simulink model "chbtask"  (R2024b)
settings: Solver=FixedStepDiscrete  StartTime=0.0  StopTime=0.2  FixedStep=5e-5  RelTol=1e-3
values from neighbouring files (symbols this model uses):
  CHB_MODE : value not decoded    [CHB_Data.sldd]
  INV120_CUURENTLOOP_KP = 2.0    [CHB_Data.sldd]
  INV120_CUURENTLOOP_KR = 5.0    [CHB_Data.sldd]
  INV120_VOLTAGELOOP_KI = 0.005    [CHB_Data.sldd]
  INV120_VOLTAGELOOP_KP = 0.5    [CHB_Data.sldd]
  INV240_VOLTAGELOOP_KI = 0.005    [CHB_Data.sldd]
  INV240_VOLTAGELOOP_KP = 0.5    [CHB_Data.sldd]
  PFC120_CUURENTLOOP_KP = 30.0    [CHB_Data.sldd]
  PFC120_CUURENTLOOP_KR = 8.0    [CHB_Data.sldd]
  PFC120_POWERLOOP_KI = 0.0001    [CHB_Data.sldd]
  PFC120_POWERLOOP_KP = 0.005    [CHB_Data.sldd]
  PFC240_CUURENTLOOP_KP = 5.0    [CHB_Data.sldd]
  PFC240_CUURENTLOOP_KR = 10.0    [CHB_Data.sldd]
  PFC240_POWERLOOP_KI = 0.0001    [CHB_Data.sldd]
  PFC240_POWERLOOP_KP = 0.005    [CHB_Data.sldd]
undefined symbols (not defined in the file or in its folder): Ii_rms, Io_rms, Io_rms_a, Io_rms_b, Vi_freq, Vi_rms, Vo_freq, Vo_freq_a, Vo_freq_b, Vo_rms, Vo_rms_a, Vo_rms_b
(part 1 of 3)
settings Model: DataDictionary=CHB_Data.sldd  Creator=licuiting  LastModifiedBy=licuiting
settings OptimizationCC: DefaultParameterBehavior=Inlined  ZeroExternalMemoryAtStartup=off  ZeroInternalMemoryAtStartup=off  OptimizeBlockOrder=speed  DifferentSizesBufferReuse=on  EfficientTunableParamExpr=on
settings DebuggingCC: ParameterTunabilityLossMsg=error
settings HardwareCC: ProdBitPerPointer=32  ProdBitPerSizeT=32  ProdBitPerPtrDiffT=32  ProdLargestAtomicInteger=Long  ProdLargestAtomicFloat=Double  ProdEndianess=BigEndian  ProdWordSize=32  ProdHWDeviceType=Freescale->32-bit PowerPC
settings ModelReferenceCC: EnableRefExpFcnMdlSchedulingChecks=on  ModelReferenceNumInstancesAllowed=Single  PropagateSignalLabelsOutOfModel=off
settings SFSimCC: MATLABDynamicMemAlloc=off
settings RTWCC: Description=Embedded Coder  SystemTargetFile=ert.tlc  GenCodeOnly=on  TemplateMakefile=ert_default_tmf  GenerateReport=on  IncludeHyperlinkInReport=on  LaunchReport=on  PortableWordSizes=on  GenerateCodeMetricsReport=on
settings CodeAppCC: IgnoreCustomStorageClasses=off  SFDataObjDesc=on  MATLABFcnDesc=on  CustomSymbolStrGlobalVar=$N$M  CustomSymbolStrType=$N$R$M  InternalIdentifier=Classic
settings ERTTargetCC: TargetLangStandard=C99 (ISO)  SuppressErrorStatus=on  SupportNonFinite=off  SupportComplex=off  ERTCustomFileTemplate=example_file_process.tlc  GlobalDataDefinition=InSourceFile  GlobalDataReference=InSourceFile  ERTFilePackagingFormat=Compact

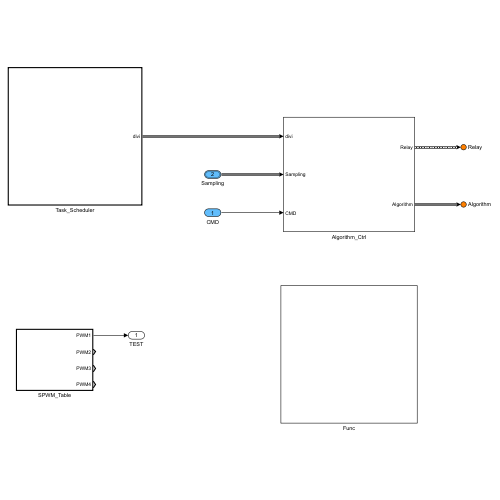
[thumbnail: Simulink's stored preview of the top-level diagram]
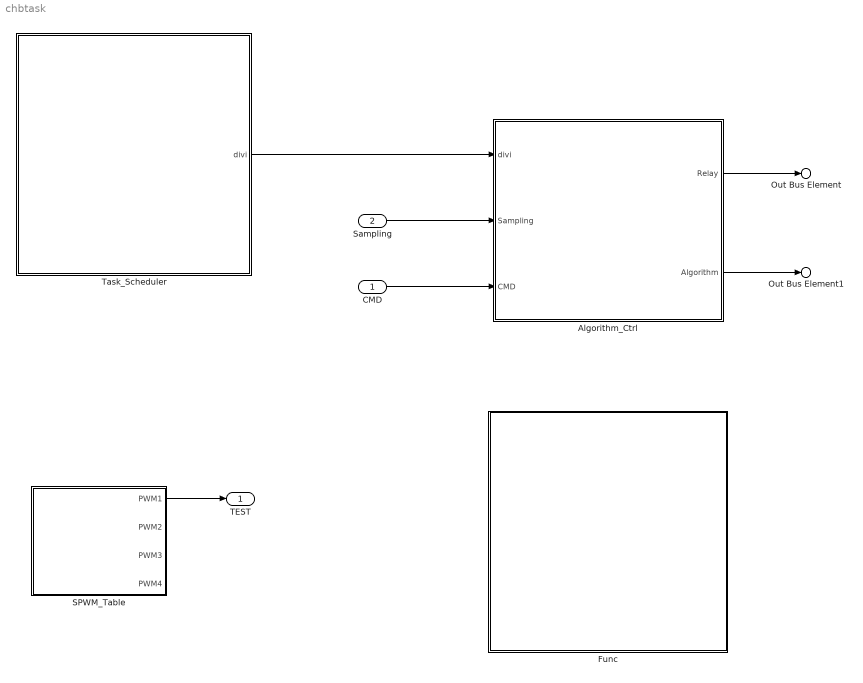
== system chbtask ==
  CMD : Inport
  Sampling : Inport  Port=2  OutDataTypeStr=Bus: Sampling_t
  Algorithm_Ctrl : Subsystem
  Func : Subsystem
  SPWM_Table : Subsystem  TreatAsAtomicUnit=on
  Task_Scheduler : Subsystem  TreatAsAtomicUnit=on
  TEST : Outport  OutDataTypeStr=single
  Out Bus Element : Outport  Port=2  PortName=Relay
  Out Bus Element1 : Outport  Port=3  PortName=Algorithm
  wires:
  Task_Scheduler/1(divi) -> Algorithm_Ctrl/1(divi)
  Sampling/1 -> Algorithm_Ctrl/2(Sampling)
  SPWM_Table/1(PWM1) -> TEST/1
  CMD/1 -> Algorithm_Ctrl/3(CMD)
  Algorithm_Ctrl/1(Relay) -> Out Bus Element/1
  Algorithm_Ctrl/2(Algorithm) -> Out Bus Element1/1

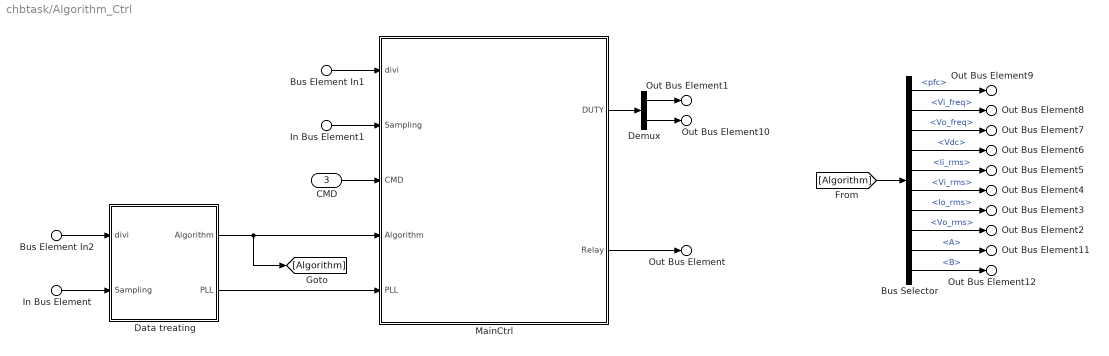
== system chbtask/Algorithm_Ctrl ==
  Bus Element In2 : Inport  PortName=divi
  Bus Element In1 : Inport  PortName=divi
  In Bus Element : Inport  Port=2  PortName=Sampling
  In Bus Element1 : Inport  Port=2  PortName=Sampling
  CMD : Inport  Port=3
  Bus Selector : BusSelector  OutputSignals=pfc,Vi_freq,Vo_freq,Vdc,Ii_rms,Vi_rms,Io_rms,Vo_rms,A,B
  Data treating : Subsystem
  Demux : Demux  Outputs=2
  MainCtrl : Subsystem
  Out Bus Element : Outport  PortName=Relay
  Out Bus Element2 : Outport  Description=输出有效值  Port=2  PortName=Algorithm  Element=Vo_rms
  Out Bus Element3 : Outport  Description=输出有效值  Port=2  PortName=Algorithm  Element=Io_rms
  Out Bus Element4 : Outport  Description=输入有效值  Port=2  PortName=Algorithm  Element=Vi_rms
  Out Bus Element5 : Outport  Description=输入有效值  Port=2  PortName=Algorithm  Element=Ii_rms
  Out Bus Element6 : Outport  Port=2  PortName=Algorithm  Element=Vdc
  Out Bus Element1 : Outport  Port=2  PortName=Algorithm  Element=duty_a
  Out Bus Element10 : Outport  Port=2  PortName=Algorithm  Element=duty_b
  Out Bus Element7 : Outport  Port=2  PortName=Algorithm  Element=Vo_freq
  Out Bus Element8 : Outport  Port=2  PortName=Algorithm  Element=Vi_freq
  Out Bus Element11 : Outport  Port=2  PortName=Algorithm  Element=A
  Out Bus Element12 : Outport  Port=2  PortName=Algorithm  Element=B
  Out Bus Element9 : Outport  Port=2  PortName=Algorithm  Element=pfc
  wires:
  Bus Element In2/1 -> Data treating/1(divi)
  In Bus Element/1 -> Data treating/2(Sampling)
  In Bus Element1/1 -> MainCtrl/2(Sampling)
  Bus Element In1/1 -> MainCtrl/1(divi)
  CMD/1 -> MainCtrl/3(CMD)
  MainCtrl/2(Relay) -> Out Bus Element/1
  Data treating/2(PLL) -> MainCtrl/5(PLL)
  Data treating/1(Algorithm) -> MainCtrl/4(Algorithm), [Algorithm]
  [Algorithm] -> Bus Selector/1
  Bus Selector/8 -> Out Bus Element2/1  "<Vo_rms>"
  Bus Selector/7 -> Out Bus Element3/1  "<Io_rms>"
  Bus Selector/6 -> Out Bus Element4/1  "<Vi_rms>"
  Bus Selector/5 -> Out Bus Element5/1  "<Ii_rms>"
  Bus Selector/4 -> Out Bus Element6/1  "<Vdc>"
  Bus Selector/3 -> Out Bus Element7/1  "<Vo_freq>"
  Bus Selector/2 -> Out Bus Element8/1  "<Vi_freq>"
  Bus Selector/1 -> Out Bus Element9/1  "<pfc>"
  MainCtrl/1(DUTY) -> Demux/1
  Demux/1 -> Out Bus Element1/1
  Demux/2 -> Out Bus Element10/1
  Bus Selector/9 -> Out Bus Element11/1  "<A>"
  Bus Selector/10 -> Out Bus Element12/1  "<B>"

== system chbtask/Func ==
  note: 踩坑：如果要重复调用函数处理不同的数据，Simulink Function内严禁出现
      | delay、积分 等考虑过去、未来时序状态参数的任何逻辑处理！！！！！！！！！
  note: 关于交流电流的控制（包括整流、逆变）
      | 目前主流方法有：
      | 旋转系(dq)：
      | 1.旋转坐标系的对q轴分量做PI控制+ 电网电压前馈 做电流环补偿
      | 静止系(αβ)：
      | 1.静止坐标系下的瞬时电流PR控制 + 电网电压前馈 做电流环补偿
      | 2.静止坐标系下的瞬时电流比例+重复控制+ 电网电压前馈 做电流环补偿
  note: 原子子系统与普通子系统的区别：
      | 普通子系统 可以在运行过程中引入外界或者被外界打断，也就是与外界信号交互能力强
      | 原子子系统 必须保证系统内部的算法全部运算完毕后，把out值传递给外部，适合运行一个完整的系统，如锁相环、SOGI、电压电流环等算法
  Rms : Subsystem  TreatAsAtomicUnit=on
  Simulink Function : Subsystem  TreatAsAtomicUnit=on
  Simulink Function1 : Subsystem  TreatAsAtomicUnit=on
  Simulink Function10 : Subsystem  TreatAsAtomicUnit=on
  Simulink Function11 : Subsystem  TreatAsAtomicUnit=on
  Simulink Function2 : Subsystem  TreatAsAtomicUnit=on
  Simulink Function3 : Subsystem  TreatAsAtomicUnit=on
  Simulink Function4 : Subsystem  TreatAsAtomicUnit=on
  Simulink Function5 : Subsystem  TreatAsAtomicUnit=on
  Simulink Function6 : Subsystem  TreatAsAtomicUnit=on
  Simulink Function7 : Subsystem  TreatAsAtomicUnit=on
  Simulink Function9 : Subsystem  TreatAsAtomicUnit=on

== system chbtask/SPWM_Table ==
  SPWM_Chart : Stateflow chart  TreatAsAtomicUnit=on
  Scope : Scope  NumInputPorts=4
  PWM1 : Outport  OutDataTypeStr=single
  PWM2 : Outport  Port=2
  PWM3 : Outport  Port=3
  PWM4 : Outport  Port=4
  wires:
  SPWM_Chart/1(PWM1) -> Scope/1, PWM1/1
  SPWM_Chart/2(PWM2) -> Scope/2, PWM2/1
  SPWM_Chart/3(PWM3) -> Scope/3, PWM3/1
  SPWM_Chart/4(PWM4) -> PWM4/1, Scope/4

== system chbtask/Task_Scheduler ==
  Chart : Stateflow chart  TreatAsAtomicUnit=on
  Chart1 : Stateflow chart  Commented=on  TreatAsAtomicUnit=on
  Scope : Scope  Commented=on
  Out Bus Element : Outport  PortName=divi  Element=1k_task1
  BusElementOut : Outport  PortName=divi  Element=1k_task2
  BusElementOut1 : Outport  PortName=divi  Element=1k_task3
  BusElementOut2 : Outport  PortName=divi  Element=1k_task4
  BusElementOut3 : Outport  PortName=divi  Element=1k_task5
  Out Bus Element1 : Outport  PortName=divi  Element=5k_task1
  Out Bus Element2 : Outport  PortName=divi  Element=5k_task2
  Out Bus Element3 : Outport  PortName=divi  Element=5k_task3
  Out Bus Element4 : Outport  PortName=divi  Element=5k_task4
  Out Bus Element5 : Outport  PortName=divi  Element=5k_task5
  Out Bus Element6 : Outport  PortName=divi  Element=10k_task1
  Out Bus Element7 : Outport  PortName=divi  Element=10k_task2
  Out Bus Element8 : Outport  PortName=divi  Element=20k_task
  wires:
  Chart/1(freq_01k_flg1()) -> Out Bus Element/1
  Chart/2(freq_01k_flg2()) -> BusElementOut/1
  Chart/3(freq_01k_flg3()) -> BusElementOut1/1
  Chart/4(freq_01k_flg4()) -> BusElementOut2/1
  Chart/5(freq_01k_flg5()) -> BusElementOut3/1
  Chart/6(freq_05k_flg1()) -> Out Bus Element1/1
  Chart/7(freq_05k_flg2()) -> Out Bus Element2/1
  Chart/8(freq_5k_flg3()) -> Out Bus Element3/1
  Chart/9(freq_5k_flg4()) -> Out Bus Element4/1
  Chart/10(freq_5k_flg5()) -> Out Bus Element5/1
  Chart/11(freq_10k_flg1()) -> Out Bus Element6/1
  Chart/12(freq_10k_flg2()) -> Out Bus Element7/1
  Chart/13(freq_20k_flg()) -> Out Bus Element8/1
  Chart1/1(out) -> Scope/1

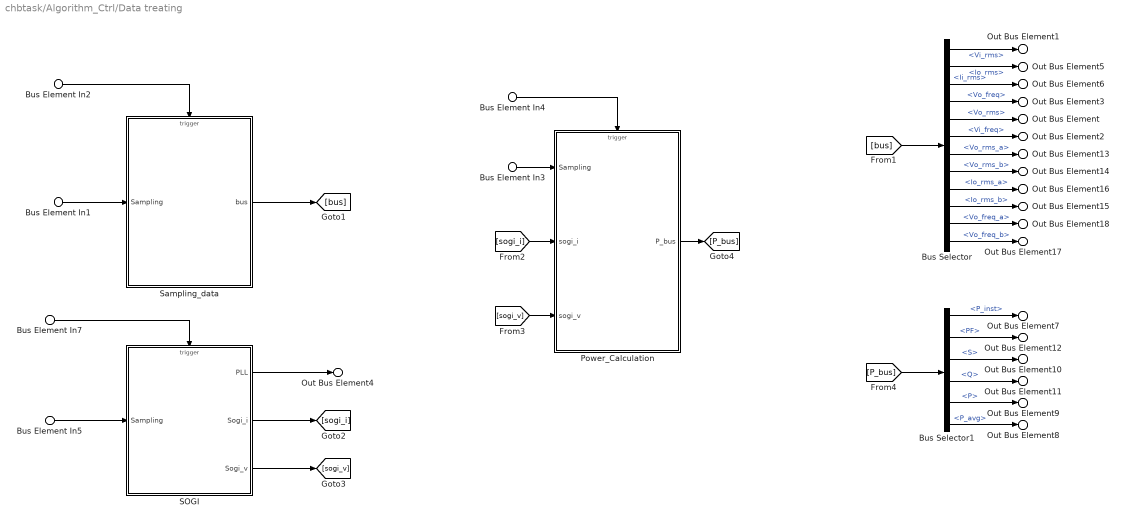
== system chbtask/Algorithm_Ctrl/Data treating ==
  Bus Element In2 : Inport  PortName=divi  Element=20k_task
  Bus Element In4 : Inport  PortName=divi  Element=1k_task1
  Bus Element In7 : Inport  PortName=divi  Element=10k_task1
  Bus Element In1 : Inport  Port=2  PortName=Sampling
  Bus Element In3 : Inport  Port=2  PortName=Sampling
  Bus Element In5 : Inport  Port=2  PortName=Sampling
  Bus Selector : BusSelector  OutputSignals=Vi_rms,Io_rms,Ii_rms,Vo_freq,Vo_rms,Vi_freq,Vo_rms_a,Vo_rms_b,Io_rms_a,Io_rms_b,Vo_freq_a,Vo_freq_b
  Bus Selector1 : BusSelector  OutputSignals=P_inst,PF,S,Q,P,P_avg
  Power_Calculation : Subsystem
  SOGI : Subsystem
  Sampling_data : Subsystem
  Out Bus Element : Outport  Description=输出有效值  PortName=Algorithm  Element=Vo_rms
  Out Bus Element5 : Outport  Description=输出有效值  PortName=Algorithm  Element=Io_rms
  Out Bus Element1 : Outport  Description=输入有效值  PortName=Algorithm  Element=Vi_rms
  Out Bus Element6 : Outport  Description=输入有效值  PortName=Algorithm  Element=Ii_rms
  Out Bus Element3 : Outport  PortName=Algorithm  Element=Vo_freq
  Out Bus Element2 : Outport  PortName=Algorithm  Element=Vi_freq
  Out Bus Element13 : Outport  PortName=Algorithm  Element=A.Vo_rms
  Out Bus Element16 : Outport  PortName=Algorithm  Element=A.Io_rms
  Out Bus Element18 : Outport  PortName=Algorithm  Element=A.Vo_freq
  Out Bus Element14 : Outport  PortName=Algorithm  Element=B.Vo_rms
  Out Bus Element15 : Outport  PortName=Algorithm  Element=B.Io_rms
  Out Bus Element17 : Outport  PortName=Algorithm  Element=B.Vo_freq
  Out Bus Element7 : Outport  Description=瞬时功率  PortName=Algorithm  Element=pfc.P_inst
  Out Bus Element8 : Outport  Description=平均功率  PortName=Algorithm  Element=pfc.P_avg
  Out Bus Element9 : Outport  Description=有功功率  PortName=Algorithm  Element=pfc.P
  Out Bus Element10 : Outport  Description=视在功率  PortName=Algorithm  Element=pfc.S
  Out Bus Element11 : Outport  Description=无功功率  PortName=Algorithm  Element=pfc.Q
  Out Bus Element12 : Outport  Description=功率因数  PortName=Algorithm  Element=pfc.PF
  Out Bus Element4 : Outport  Port=2  PortName=PLL
  wires:
  Bus Element In2/1 -> Sampling_data/Trigger
  Bus Element In4/1 -> Power_Calculation/Trigger
  Bus Element In1/1 -> Sampling_data/1(Sampling)
  Bus Element In3/1 -> Power_Calculation/1(Sampling)
  Bus Element In7/1 -> SOGI/Trigger
  Bus Element In5/1 -> SOGI/1(Sampling)
  SOGI/1(PLL) -> Out Bus Element4/1
  [bus] -> Bus Selector/1
  Bus Selector/4 -> Out Bus Element3/1  "<Vo_freq>"
  Bus Selector/1 -> Out Bus Element1/1  "<Vi_rms>"
  Bus Selector/2 -> Out Bus Element5/1  "<Io_rms>"
  Bus Selector/6 -> Out Bus Element2/1  "<Vi_freq>"
  Bus Selector/3 -> Out Bus Element6/1  "<Ii_rms>"
  Bus Selector/5 -> Out Bus Element/1  "<Vo_rms>"
  SOGI/2(Sogi_i) -> [sogi_i]
  SOGI/3(Sogi_v) -> [sogi_v]
  [sogi_i] -> Power_Calculation/2(sogi_i)
  [sogi_v] -> Power_Calculation/3(sogi_v)
  Power_Calculation/1(P_bus) -> [P_bus]
  [P_bus] -> Bus Selector1/1
  Bus Selector1/1 -> Out Bus Element7/1  "<P_inst>"
  Bus Selector1/3 -> Out Bus Element10/1  "<S>"
  Bus Selector1/4 -> Out Bus Element11/1  "<Q>"
  Bus Selector1/2 -> Out Bus Element12/1  "<PF>"
  Bus Selector1/5 -> Out Bus Element9/1  "<P>"
  Bus Selector1/6 -> Out Bus Element8/1  "<P_avg>"
  Sampling_data/1(bus) -> [bus]
  Bus Selector/7 -> Out Bus Element13/1  "<Vo_rms_a>"
  Bus Selector/8 -> Out Bus Element14/1  "<Vo_rms_b>"
  Bus Selector/9 -> Out Bus Element16/1  "<Io_rms_a>"
  Bus Selector/10 -> Out Bus Element15/1  "<Io_rms_b>"
  Bus Selector/11 -> Out Bus Element18/1  "<Vo_freq_a>"
  Bus Selector/12 -> Out Bus Element17/1  "<Vo_freq_b>"

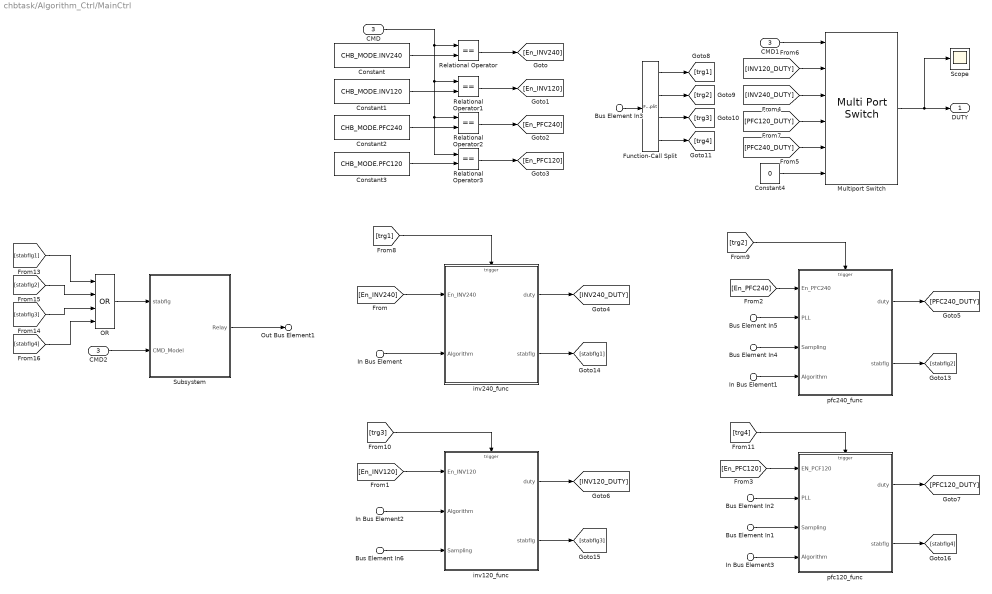
== system chbtask/Algorithm_Ctrl/MainCtrl ==
  Bus Element In3 : Inport  PortName=divi  Element=10k_task2
  Bus Element In4 : Inport  Port=2  PortName=Sampling
  Bus Element In1 : Inport  Port=2  PortName=Sampling
  Bus Element In6 : Inport  Port=2  PortName=Sampling
  CMD : Inport  Port=3
  In Bus Element{,1..3} (4 alike) : Inport  Port=4  PortName=Algorithm
  Bus Element In5 : Inport  Port=5  PortName=PLL
  Bus Element In2 : Inport  Port=5  PortName=PLL
  CMD1 : InportShadow  Port=3
  CMD2 : InportShadow  Port=3
  Constant : Constant  Value=CHB_MODE.INV240  OutDataTypeStr=Enum: CHB_MODE
  Constant1 : Constant  Value=CHB_MODE.INV120  OutDataTypeStr=Enum: CHB_MODE
  Constant2 : Constant  Value=CHB_MODE.PFC240  OutDataTypeStr=Enum: CHB_MODE
  Constant3 : Constant  Value=CHB_MODE.PFC120  OutDataTypeStr=Enum: CHB_MODE
  Constant4 : Constant  Value=0
  Function-Call Split : FunctionCallSplit  IconShape=distinctive  NumOutputPorts=4  OutputPortLayout=default
  Multiport Switch : MultiPortSwitch  DataPortOrder=Specify indices  Inputs=4  DataPortIndices={CHB_MODE.INV120,CHB_MODE.INV240,CHB_MODE.PFC120,CHB_MODE.PFC240,CHB_MODE.STANDBY}  OutDataTypeStr=single  SaturateOnIntegerOverflow=off  InputSameDT=off
  OR : Logic  Operator=OR  Inputs=4  IconShape=distinctive  AllPortsSameDT=off  OutDataTypeStr=boolean
  Relational Operator{,1..3} (4 alike) : RelationalOperator  Operator===  OutDataTypeStr=boolean  RndMeth=Simplest  InputSameDT=off
  Scope : Scope
  Subsystem : Subsystem
  inv120_func : Subsystem
  inv240_func : Subsystem
  pfc120_func : Subsystem
  pfc240_func : Subsystem
  DUTY : Outport  OutDataTypeStr=single  PortDimensions=[1 2]  VectorParamsAs1DForOutWhenUnconnected=off
  Out Bus Element1 : Outport  Port=2  PortName=Relay
  wires:
  CMD/1 -> Relational Operator3/1, Relational Operator2/1, Relational Operator1/1, Relational Operator/1
  Relational Operator2/1 -> [En_PFC240]
  Relational Operator3/1 -> [En_PFC120]
  Constant/1 -> Relational Operator/2
  Constant3/1 -> Relational Operator3/2
  Constant1/1 -> Relational Operator1/2
  Relational Operator1/1 -> [En_INV120]
  Relational Operator/1 -> [En_INV240]
  Constant2/1 -> Relational Operator2/2
  CMD1/1 -> Multiport Switch/1
  [INV240_DUTY] -> Multiport Switch/3
  [PFC240_DUTY] -> Multiport Switch/5
  [INV120_DUTY] -> Multiport Switch/2
  [PFC120_DUTY] -> Multiport Switch/4
  Constant4/1 -> Multiport Switch/6
  Multiport Switch/1 -> DUTY/1, Scope/1
  inv240_func/1(duty) -> [INV240_DUTY]
  [En_INV240] -> inv240_func/1(En_INV240)
  [En_INV120] -> inv120_func/1(En_INV120)
  inv120_func/1(duty) -> [INV120_DUTY]
  pfc120_func/1(duty) -> [PFC120_DUTY]
  [En_PFC120] -> pfc120_func/1(EN_PCF120)
  [En_PFC240] -> pfc240_func/1(En_PFC240)
  pfc240_func/1(duty) -> [PFC240_DUTY]
  Bus Element In3/1 -> Function-Call Split/1
  Function-Call Split/1 -> [trg1]
  Function-Call Split/2 -> [trg2]
  Function-Call Split/4 -> [trg4]
  Function-Call Split/3 -> [trg3]
  [trg1] -> inv240_func/Trigger
  [trg2] -> pfc240_func/Trigger
  [trg3] -> inv120_func/Trigger
  [trg4] -> pfc120_func/Trigger
  Bus Element In5/1 -> pfc240_func/2(PLL)
  CMD2/1 -> Subsystem/2(CMD_Model)
  Subsystem/1(Relay) -> Out Bus Element1/1
  pfc240_func/2(stabflg) -> [stabflg2]
  inv240_func/2(stabflg) -> [stabflg1]
  inv120_func/2(stabflg) -> [stabflg3]
  pfc120_func/2(stabflg) -> [stabflg4]
  OR/1 -> Subsystem/1(stabflg)
  [stabflg2] -> OR/2
  [stabflg3] -> OR/3
  [stabflg4] -> OR/4
  [stabflg1] -> OR/1
  Bus Element In4/1 -> pfc240_func/3(Sampling)
  In Bus Element/1 -> inv240_func/2(Algorithm)
  In Bus Element1/1 -> pfc240_func/4(Algorithm)
  In Bus Element2/1 -> inv120_func/2(Algorithm)
  Bus Element In2/1 -> pfc120_func/2(PLL)
  Bus Element In1/1 -> pfc120_func/3(Sampling)
  In Bus Element3/1 -> pfc120_func/4(Algorithm)
  Bus Element In6/1 -> inv120_func/3(Sampling)

== system chbtask/Func/Rms ==
  note: 大学以前的有效值采样是基于已知采样周期、基波频率，采样点数三个已知条件计算有效值的，这种采样是默认了采样波是平滑稳定的，粗暴地代入已知条件 不具有判断采样波是否正常的能力，无法检测输入异常与相关保护 ，实际上，基波频率、有效值都应该是计算出来的。采样点数有上下限的限制，允许有一定的误差，只有ADC的采样周期是已知的
  f : TriggerPort  TriggerType=function-call  IsSimulinkFunction=on  FunctionName=Rms  FunctionVisibility=scoped  VariantControl=(inherit)
  RMS : MATLAB Function  TreatAsAtomicUnit=on
  Fs : ArgIn  DisableCoverage=on  OutDataTypeStr=single  ArgumentName=Fs
  X_data : ArgIn  DisableCoverage=on  Port=2  OutDataTypeStr=single  ArgumentName=X_data
  limit_cnt : ArgIn  DisableCoverage=on  Port=3  OutDataTypeStr=single  PortDimensions=[1,2]  ArgumentName=limit_cnt
  pre_data : ArgIn  DisableCoverage=on  Port=4  OutDataTypeStr=single  PortDimensions=[1,5]  ArgumentName=pre_data
  X_rms : ArgOut  DisableCoverage=on  OutDataTypeStr=single  ArgumentName=X_rms
  X_freq : ArgOut  DisableCoverage=on  Port=2  OutDataTypeStr=single  ArgumentName=X_freq
  out_data : ArgOut  DisableCoverage=on  Port=3  OutDataTypeStr=single  PortDimensions=[1,5]  ArgumentName=out_data
  wires:
  Fs/1 -> RMS/1(Fs)
  X_data/1 -> RMS/2(X_data)
  limit_cnt/1 -> RMS/3(limit_cnt)
  pre_data/1 -> RMS/4(pre_data)
  RMS/1(X_rms) -> X_rms/1
  RMS/2(X_freq) -> X_freq/1
  RMS/3(out_data) -> out_data/1

== system chbtask/Func/Simulink Function ==
  note: 缺点：直接暴力带入双线性差分公式需要涉及系统h(k-1)和h(k-2)的参数，
      | 系统不建议用上上一个甚至更上的输出值，
      | 时效性高才是最好的， 代数过多，算法复杂。 但是Tustin的精度和稳定性很高，算力充足情况下还是非常推荐使用的。
  note: alpha输出： $H_{\alpha}(s) = \frac{k{\omega}s}{s^2+k{\omega}s+{\omega}^2}$
      | beta输出： $H_{\beta}(s)=\frac{k{\omega}^2}{s^2+k{\omega}s + {\omega}^2}$
  Sogi_Tustin : TriggerPort  TriggerType=function-call  IsSimulinkFunction=on  FunctionName=Sogi_Tustin  FunctionVisibility=scoped  VariantControl=(inherit)
  Chart : Stateflow chart  TreatAsAtomicUnit=on
  uk : ArgIn  DisableCoverage=on  OutDataTypeStr=single  ArgumentName=uk
  freq : ArgIn  DisableCoverage=on  Port=2  OutDataTypeStr=single  ArgumentName=freq
  k : ArgIn  DisableCoverage=on  Port=3  OutDataTypeStr=single  ArgumentName=k
  T : ArgIn  DisableCoverage=on  Port=4  OutDataTypeStr=single  ArgumentName=T
  alpha : ArgOut  DisableCoverage=on  OutDataTypeStr=single  ArgumentName=alpha
  beta : ArgOut  DisableCoverage=on  Port=2  OutDataTypeStr=single  ArgumentName=beta
  wires:
  T/1 -> Chart/4(T)  "系统周期"
  uk/1 -> Chart/1(uk)  "输入信号"
  k/1 -> Chart/3(k)  "阻尼系数"
  freq/1 -> Chart/2(wt)  "电网频率"
  Chart/1(alpha) -> alpha/1
  Chart/2(beta) -> beta/1

== system chbtask/Func/Simulink Function1 ==
  fault_detect : TriggerPort  TriggerType=function-call  IsSimulinkFunction=on  FunctionName=fault_detect  FunctionVisibility=scoped  VariantControl=(inherit)
  Delay : Delay  DelayLength=1  InputProcessing=Columns as channels (frame based)
  Delay1 : Delay  DelayLength=1  InputProcessing=Columns as channels (frame based)
  MATLAB Function : MATLAB Function  TreatAsAtomicUnit=on
  fault_in : ArgIn  DisableCoverage=on  OutDataTypeStr=boolean  ArgumentName=fault_in
  recover_in : ArgIn  DisableCoverage=on  Port=2  OutDataTypeStr=boolean  ArgumentName=recover_in
  fault_cnt : ArgIn  DisableCoverage=on  Port=3  OutDataTypeStr=int16  ArgumentName=fault_cnt
  recover_cnt : ArgIn  DisableCoverage=on  Port=4  OutDataTypeStr=int16  ArgumentName=recover_cnt
  lock_en : ArgIn  DisableCoverage=on  Port=5  OutDataTypeStr=boolean  ArgumentName=lock_en
  fault_en : ArgOut  DisableCoverage=on  OutDataTypeStr=uint32  ArgumentName=fault_en
  wires:
  MATLAB Function/1(fault_en) -> Delay1/1, fault_en/1
  fault_in/1 -> MATLAB Function/1(fault_in)
  recover_in/1 -> MATLAB Function/2(recover_in)
  fault_cnt/1 -> MATLAB Function/3(fault_cnt)
  recover_cnt/1 -> MATLAB Function/4(recover_cnt)
  lock_en/1 -> MATLAB Function/5(lock_en)
  MATLAB Function/2(cnt) -> Delay/1
  Delay/1 -> MATLAB Function/7("cnt ")
  Delay1/1 -> MATLAB Function/6("fault_en ")

== system chbtask/Func/Simulink Function10 ==
  note: 无功功率: $q=u_{\alpha}i_{\beta}-u_{\beta}i_{\alpha}$ q有时候定义是反相的，根据需求决定
      | 有功功率: $p=u_{\alpha}i_{\alpha}+u_{\beta}i_{\beta}$
  ctrl_pq : TriggerPort  TriggerType=function-call  IsSimulinkFunction=on  FunctionName=ctrl_pq  FunctionVisibility=scoped  VariantControl=(inherit)
  Chart : Stateflow chart  TreatAsAtomicUnit=on
  alpha : ArgIn  DisableCoverage=on  OutDataTypeStr=single  PortDimensions=[1 2]  ArgumentName=alpha
  beta : ArgIn  DisableCoverage=on  Port=2  OutDataTypeStr=single  PortDimensions=[1 2]  ArgumentName=beta
  q : ArgOut  DisableCoverage=on  OutDataTypeStr=single  ArgumentName=q
  p : ArgOut  DisableCoverage=on  Port=2  OutDataTypeStr=single  ArgumentName=p
  wires:
  alpha/1 -> Chart/1(alpha)  "[ua  ia]"
  beta/1 -> Chart/2(beta)  "[ub  ib]"
  Chart/1(q) -> q/1
  Chart/2(p) -> p/1

== system chbtask/Func/Simulink Function11 ==
  limit : TriggerPort  TriggerType=function-call  IsSimulinkFunction=on  FunctionName=limit  FunctionVisibility=scoped  VariantControl=(inherit)
  Chart : Stateflow chart  TreatAsAtomicUnit=on
  u : ArgIn  DisableCoverage=on  OutDataTypeStr=single  ArgumentName=input
  u1 : ArgIn  DisableCoverage=on  Port=2  OutDataTypeStr=single  PortDimensions=[1 2]  ArgumentName=limit
  y : ArgOut  DisableCoverage=on  OutDataTypeStr=single  ArgumentName=out
  wires:
  Chart/1(out) -> y/1
  u1/1 -> Chart/2(limit)  "[min max]"
  u/1 -> Chart/1(input)

== system chbtask/Func/Simulink Function2 ==
  note: alpha输出： $H_{\alpha}(s) = \frac{k{\omega}s}{s^2+k{\omega}s+{\omega}^2}$$
      | beta输出： $H_{\beta}(s)=\frac{k{\omega}^2}{s^2+k{\omega}s + {\omega}^2}$$
  note: 缺点：直接暴力带入后向差分公式需要涉及系统h(k-1)和h(k-2)的参数，
      | 系统不建议用上上一个甚至更上的输出值，
      | 时效性高才是最好的， 代数过多，算法复杂
  Sogi_Back : TriggerPort  TriggerType=function-call  IsSimulinkFunction=on  FunctionName=Sogi_Back  FunctionVisibility=scoped  VariantControl=(inherit)
  Chart : Stateflow chart  TreatAsAtomicUnit=on
  uk : ArgIn  DisableCoverage=on  OutDataTypeStr=single  ArgumentName=uk
  freq : ArgIn  DisableCoverage=on  Port=2  OutDataTypeStr=single  ArgumentName=freq
  k : ArgIn  DisableCoverage=on  Port=3  OutDataTypeStr=single  ArgumentName=k
  T : ArgIn  DisableCoverage=on  Port=4  OutDataTypeStr=single  ArgumentName=T
  alpha : ArgOut  DisableCoverage=on  OutDataTypeStr=single  ArgumentName=alpha
  beta : ArgOut  DisableCoverage=on  Port=2  OutDataTypeStr=single  ArgumentName=beta
  wires:
  freq/1 -> Chart/2(wt)  "电网频率"
  k/1 -> Chart/3(k)  "阻尼系数"
  T/1 -> Chart/4(T)  "系统周期"
  uk/1 -> Chart/1(uk)  "输入信号"
  Chart/1(alpha) -> alpha/1
  Chart/2(beta) -> beta/1

== system chbtask/Func/Simulink Function3 ==
  note: alpha输出： $H_{\alpha}(s) = \frac{k{\omega}s}{s^2+k{\omega}s+{\omega}^2}$
      | beta输出： $H_{\beta}(s)=\frac{k{\omega}^2}{s^2+k{\omega}s + {\omega}^2}$
      | s^2是二阶微分算子，这个系统是二阶系统，
      | 针对 高频系统（采样>20k） ，前向欧拉 状态空间 法最简单有效
      | 为什么不能直接用s=(z-1)/T（包括双线性、后向差分）暴力带入？求出后的式子有k-2以上的代数，且前向差分不适用直接带入二阶系统。
      | 先求出状态方程公式降阶，再离散，适用于大多数电力电子算法。
      | 状态方程针对两个及以上的输出，从系统的角度而言这些输出具有很强的关联性，直接暴力带入推导各输出会显得像是各干各的。
      | 求输入、输出时域表达式-->输入、输出状态方程-->前向欧拉离散化 的步骤可大幅度减少算力， 先前推导的卡尔曼滤波也是 先求状态方程再离散（且离散也是前向欧拉） 的
      | 这种离散化方式被称之为 ZOH(零阶保持器)
  Sogi_ZOH : TriggerPort  TriggerType=function-call  IsSimulinkFunction=on  FunctionName=Sogi_ZOH  FunctionVisibility=scoped  VariantControl=(inherit)
  Chart : Stateflow chart  TreatAsAtomicUnit=on
  uk : ArgIn  DisableCoverage=on  OutDataTypeStr=single  ArgumentName=uk
  freq : ArgIn  DisableCoverage=on  Port=2  OutDataTypeStr=single  ArgumentName=freq
  T : ArgIn  DisableCoverage=on  Port=3  OutDataTypeStr=single  ArgumentName=T
  alpha1 : ArgIn  DisableCoverage=on  Port=4  OutDataTypeStr=single  ArgumentName=alpha1
  beta1 : ArgIn  DisableCoverage=on  Port=5  OutDataTypeStr=single  ArgumentName=beta1
  alpha : ArgOut  DisableCoverage=on  OutDataTypeStr=single  ArgumentName=alpha
  beta : ArgOut  DisableCoverage=on  Port=2  OutDataTypeStr=single  ArgumentName=beta
  wires:
  Chart/1(alpha) -> alpha/1
  Chart/2(beta) -> beta/1
  uk/1 -> Chart/1(uk)  "输入信号"
  T/1 -> Chart/3(T)  "系统周期"
  freq/1 -> Chart/2(wt)  "电网频率"
  alpha1/1 -> Chart/4(alpha_1)  "y_a(k-1)"
  beta1/1 -> Chart/5(beta_1)  "y_b(k-1)"

== system chbtask/Func/Simulink Function4 ==
  note: 由于有delay、微分等操作， 禁止重复调用此函数处理不同的数据
  note: 输入标幺化
  note: $u_\beta$
  note: 取模方法3
  note: 取模方法2
  note: 取模方法1
  note: αβ静态坐标轴→DQ动态坐标轴
      | 为什么要做park变换？因为αβ是交流量，瞬时值是变换的，在αβ静态坐标轴中，Uα与Uβ的大小在时刻变化，而park变换后DQ的模是固定的，即|Ud|与|Uq|是静止的。所以除了锁相环以外，DQ解耦也多用于将交流量转换为直流量便于PI控制，在三相并网逆变器中，电流DQ解耦，d轴电流控制有功功率，q轴电流控制无功功率，可实现单位功率因数或无功补偿。
      | 在初等数学中，在xy坐标轴中，一个从0点出发的向量，已知它的模为k，它映射在x轴上的长度为x=k*cosθ，在y轴上的长度为y=k*sinθ。
      | 所以αβ分解到D、Q轴之后，αβ是已知变量，为了确保|Ud|与|Uq|是静止不动的，就只有θ一个变量，而这个θ就导致DQ坐标轴旋转了起来。
      | 利用PI调节器将Q轴分量控制为0，就可以实现相位跟踪(锁相)
      | Q = -α×sinθ + β×cosθ
      | D = β×sinθ + α×cosθ
  note: $u_\alpha$
  note: 输入标幺化
  PLL : TriggerPort  TriggerType=function-call  IsSimulinkFunction=on  FunctionName=PLL  FunctionVisibility=scoped  VariantControl=(inherit)
  Add : Sum
  Chart : Stateflow chart  TreatAsAtomicUnit=on
  Chart1 : Stateflow chart  TreatAsAtomicUnit=on
  Chart2 : Stateflow chart  Commented=on  TreatAsAtomicUnit=on
  Constant : Constant  Commented=on  Value=2*pi  OutDataTypeStr=single
  Cos : Trigonometry  Operator=cos
  Delay : Delay  DelayLength=1  InputProcessing=Columns as channels (frame based)
  Gain : Gain  Gain=2*pi  OutDataTypeStr=single
  Gain1 : Gain  Gain=2e-4  OutDataTypeStr=single
  Minus : Sum  Inputs=+-  OutDataTypeStr=single  AccumDataTypeStr=single
  Mod : Math  Commented=on  Operator=mod
  Product : Product  OutDataTypeStr=single
  Product1 : Product  OutDataTypeStr=single
  Sin : Trigonometry
  Sum of Elements : Sum  Commented=on  Inputs=+
  alpha : ArgIn  DisableCoverage=on  OutDataTypeStr=single  ArgumentName=alpha
  beta : ArgIn  DisableCoverage=on  Port=2  OutDataTypeStr=single  ArgumentName=beta
  Kp : ArgIn  DisableCoverage=on  Port=3  OutDataTypeStr=single  ArgumentName=Kp
  Ki : ArgIn  DisableCoverage=on  Port=4  OutDataTypeStr=single  ArgumentName=Ki
  freq : ArgIn  DisableCoverage=on  Port=5  OutDataTypeStr=single  ArgumentName=freq
  theta : ArgOut  DisableCoverage=on  OutDataTypeStr=single  ArgumentName=theta
  cosine : ArgOut  DisableCoverage=on  Port=2  OutDataTypeStr=single  ArgumentName=cosine
  sine : ArgOut  DisableCoverage=on  Port=3  OutDataTypeStr=single  ArgumentName=sine
  wires:
  Delay/1 -> Cos/1, Sin/1
  Cos/1 -> Product/2, cosine/1
  Sin/1 -> sine/1, Product1/2
  Product/1 -> Minus/1
  Product1/1 -> Minus/2
  Minus/1 -> Chart1/3(error)  "Q轴分量"
  Ki/1 -> Chart1/2(Ki)
  Kp/1 -> Chart1/1(Kp)
  freq/1 -> Gain/1
  alpha/1 -> Product1/1
  beta/1 -> Product/1
  Chart1/1(out) -> Add/2
  Gain/1 -> Add/1  "引入前馈控制"
  Sum of Elements/1 -> Mod/1  "这里一直累加会溢出pass"
  Constant/1 -> Mod/2
  Gain1/1 -> Chart/1(uk)
  Add/1 -> Gain1/1
  Chart/1(theta) -> Delay/1, theta/1

== system chbtask/Func/Simulink Function5 ==
  note: $G(S) = K_p + \frac{K_i}{s}$
      | y(k) = p*e(k) + i * ∑ e(k)
  PI_Ctrl : TriggerPort  TriggerType=function-call  IsSimulinkFunction=on  FunctionName=PI_Ctrl  FunctionVisibility=scoped  VariantControl=(inherit)
  Chart : Stateflow chart  TreatAsAtomicUnit=on
  error : ArgIn  DisableCoverage=on  OutDataTypeStr=single  ArgumentName=error
  err_sum : ArgIn  DisableCoverage=on  Port=2  OutDataTypeStr=single  ArgumentName=err_sum
  Kp : ArgIn  DisableCoverage=on  Port=3  OutDataTypeStr=single  ArgumentName=Kp
  Ki : ArgIn  DisableCoverage=on  Port=4  OutDataTypeStr=single  ArgumentName=Ki
  out_limit : ArgIn  DisableCoverage=on  Port=5  OutDataTypeStr=single  PortDimensions=[1 2]  ArgumentName=out_limit
  PI_out : ArgOut  DisableCoverage=on  OutDataTypeStr=single  ArgumentName=PI_out
  wires:
  error/1 -> Chart/1(error)  "误差=目标值-实际值"
  Kp/1 -> Chart/3(Kp)
  Ki/1 -> Chart/4(Ki)
  Chart/1(out) -> PI_out/1
  out_limit/1 -> Chart/5(limit)  "输出限幅[max min]"
  err_sum/1 -> Chart/2(e_sum)

== system chbtask/Func/Simulink Function6 ==
  note: 变步长----扰动观测法
  MPPT : TriggerPort  TriggerType=function-call  IsSimulinkFunction=on  FunctionName=MPPT  FunctionVisibility=scoped  VariantControl=(inherit)
  Chart1 : Stateflow chart  TreatAsAtomicUnit=on
  P : ArgIn  DisableCoverage=on  OutDataTypeStr=single  ArgumentName=U_step
  Urms : ArgIn  DisableCoverage=on  Port=2  OutDataTypeStr=single  ArgumentName=Urms
  Irms : ArgIn  DisableCoverage=on  Port=3  OutDataTypeStr=single  ArgumentName=Irms
  y : ArgOut  DisableCoverage=on  OutDataTypeStr=single  ArgumentName=Uref
  wires:
  P/1 -> Chart1/3(Ustep)
  Irms/1 -> Chart1/2(Ik)
  Urms/1 -> Chart1/1(Uk)
  Chart1/1(Uref) -> y/1

== system chbtask/Func/Simulink Function7 ==
  note: 理想： $G(s)=K_p+ \frac{K_rs}{s^2+\omega^2}$
      | 实际： $G(s)=K_p+ \frac{2\omega_c K_rs}{s^2+2\omega_cs + \omega^2}$
      | 是一个带通滤波器，ω0：基波 ωc:带宽谐波(±1Hz)
  note: PR比例谐振器
      | 在电网双闭环控制中，PI常用于控制电流内环，PI在控制交流电流时，需要把其静态的αβ量进行dq解耦，转变为直流量。而对于PR而言，PR是可以在αβ坐标轴下实现对交流信号的无精差跟踪器，通过在谐振频率处提供无穷大的增益，实现对基波、谐波等特定频率正弦信号的零稳态误差控制。
      | 实际工程中，dq+PI和αβ+PR是两大主流电流控制方案，根据具体的环境与控制复杂度选择不同的主控方案。
      | 三相系统常用dq+PI，单相系统常用PR
      | 关于PR的离散化，PR是属于单输入单输出系统(SISO)推荐用 Tustin 或者 零极点匹配法 效果最佳。
      | 但是ZOH的离散化结果太过于复杂了，这里选择Tustin
      | 且只针对R部分做离散调节
  R_Ctrl : TriggerPort  TriggerType=function-call  IsSimulinkFunction=on  FunctionName=R_Ctrl  FunctionVisibility=scoped  VariantControl=(inherit)
  R : Stateflow chart  TreatAsAtomicUnit=on
  Ts : ArgIn  DisableCoverage=on  OutDataTypeStr=single  ArgumentName=Ts
  Kr : ArgIn  DisableCoverage=on  Port=2  OutDataTypeStr=single  ArgumentName=Kr
  uk : ArgIn  DisableCoverage=on  Port=3  OutDataTypeStr=single  ArgumentName=uk
  freq0 : ArgIn  DisableCoverage=on  Port=4  OutDataTypeStr=single  ArgumentName=freq0
  freqc : ArgIn  DisableCoverage=on  Port=5  OutDataTypeStr=single  ArgumentName=freqc
  R_out : ArgOut  DisableCoverage=on  OutDataTypeStr=single  ArgumentName=R_out
  wires:
  Ts/1 -> R/1(Ts)
  uk/1 -> R/3(uk)
  freq0/1 -> R/4(freq0)
  freqc/1 -> R/5(freqc)
  Kr/1 -> R/2(Kr)
  R/1(yk) -> R_out/1

== system chbtask/Func/Simulink Function9 ==
  note: 一阶滤波：
      | $Y(k) = \alpha X(k)+(1-\alpha)Y(k-1)$
  lpf : TriggerPort  TriggerType=function-call  IsSimulinkFunction=on  FunctionName=lpf  FunctionVisibility=scoped  VariantControl=(inherit)
  Chart : Stateflow chart  TreatAsAtomicUnit=on
  u : ArgIn  DisableCoverage=on  OutDataTypeStr=single  ArgumentName=input
  u1 : ArgIn  DisableCoverage=on  Port=2  OutDataTypeStr=single  ArgumentName=factor
  u2 : ArgIn  DisableCoverage=on  Port=3  OutDataTypeStr=single  ArgumentName=out_pre
  y : ArgOut  DisableCoverage=on  OutDataTypeStr=single  ArgumentName=out
  wires:
  u/1 -> Chart/1(input)
  u1/1 -> Chart/2(factor)
  Chart/1(out) -> y/1
  u2/1 -> Chart/3(out_pre)

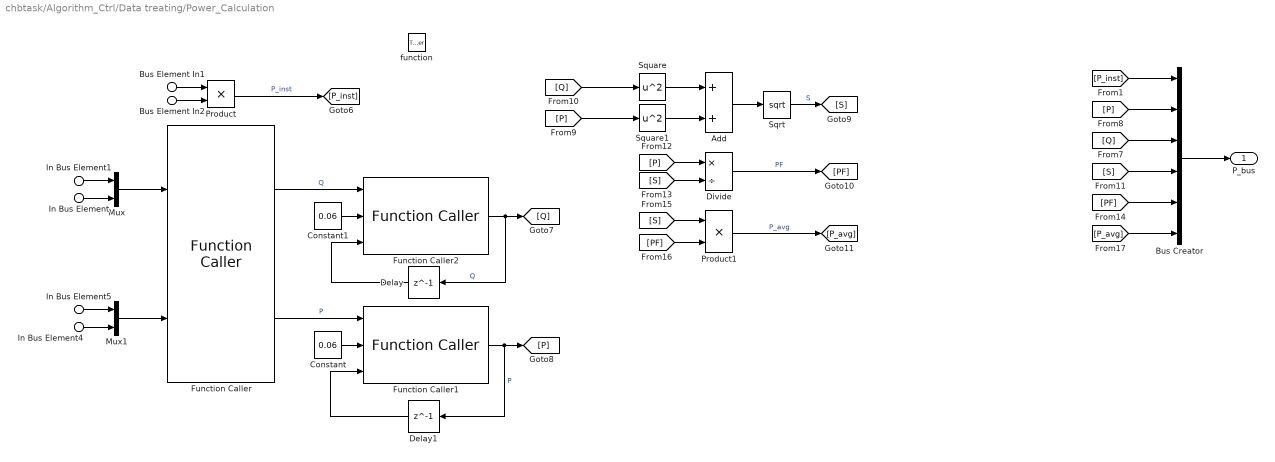
== system chbtask/Algorithm_Ctrl/Data treating/Power_Calculation ==
  Bus Element In1 : Inport  PortName=Sampling  Element=AC_in.Vgrid
  Bus Element In2 : Inport  PortName=Sampling  Element=AC_in.Igrid
  In Bus Element : Inport  Port=2  PortName=sogi_i  Element=alpha
  In Bus Element4 : Inport  Port=2  PortName=sogi_i  Element=beta
  In Bus Element1 : Inport  Port=3  PortName=sogi_v  Element=alpha
  In Bus Element5 : Inport  Port=3  PortName=sogi_v  Element=beta
  function : TriggerPort  TriggerType=function-call  VariantControl=(inherit)
  Add : Sum  OutDataTypeStr=single  AccumDataTypeStr=single
  Bus Creator : BusCreator  Inputs=6
  Constant : Constant  Value=0.06  OutDataTypeStr=single
  Constant1 : Constant  Value=0.06  OutDataTypeStr=single
  Delay : Delay  DelayLength=1  InputProcessing=Columns as channels (frame based)
  Delay1 : Delay  DelayLength=1  InputProcessing=Columns as channels (frame based)
  Divide : Product  Inputs=*/  OutDataTypeStr=single
  Function Caller : FunctionCaller  FunctionPrototype=[q,p] = Func.ctrl_pq(alpha,beta)  InputArgumentSpecifications=<Enter example>  OutputArgumentSpecifications=<Enter example>
  Function Caller1 : FunctionCaller  FunctionPrototype=out = Func.lpf(input,factor,out_pre)  InputArgumentSpecifications=<Enter example>  OutputArgumentSpecifications=<Enter example>
  Function Caller2 : FunctionCaller  FunctionPrototype=out = Func.lpf(input,factor,out_pre)  InputArgumentSpecifications=<Enter example>  OutputArgumentSpecifications=<Enter example>
  Mux : Mux  Inputs=2
  Mux1 : Mux  Inputs=2
  Product : Product  OutDataTypeStr=single
  Product1 : Product  OutDataTypeStr=single
  Sqrt : Sqrt  OutDataTypeStr=single
  Square : Math  Operator=square  OutDataTypeStr=single
  Square1 : Math  Operator=square  OutDataTypeStr=single
  P_bus : Outport
  wires:
  Bus Element In1/1 -> Product/1
  Bus Element In2/1 -> Product/2
  In Bus Element/1 -> Mux/2
  In Bus Element1/1 -> Mux/1
  Mux1/1 -> Function Caller/2
  In Bus Element4/1 -> Mux1/2
  In Bus Element5/1 -> Mux1/1
  Product/1 -> [P_inst]  "P_inst"
  [Q] -> Square/1
  [P] -> Square1/1
  Square/1 -> Add/1
  Square1/1 -> Add/2
  Add/1 -> Sqrt/1
  Sqrt/1 -> [S]  "S"
  [P] -> Divide/1
  Divide/1 -> [PF]  "PF"
  [P_inst] -> Bus Creator/1
  [P] -> Bus Creator/2
  [Q] -> Bus Creator/3
  [S] -> Bus Creator/4
  [PF] -> Bus Creator/5
  Bus Creator/1 -> P_bus/1
  [S] -> Product1/1
  [PF] -> Product1/2
  Product1/1 -> [P_avg]  "P_avg"
  [P_avg] -> Bus Creator/6
  [S] -> Divide/2
  Function Caller1/1 -> Delay1/1, [P]  "P"
  Function Caller/2 -> Function Caller1/1  "P"
  Function Caller/1 -> Function Caller2/1  "Q"
  Function Caller2/1 -> Delay/1, [Q]  "Q"
  Mux/1 -> Function Caller/1
  Delay1/1 -> Function Caller1/3
  Delay/1 -> Function Caller2/3
  Constant1/1 -> Function Caller2/2
  Constant/1 -> Function Caller1/2

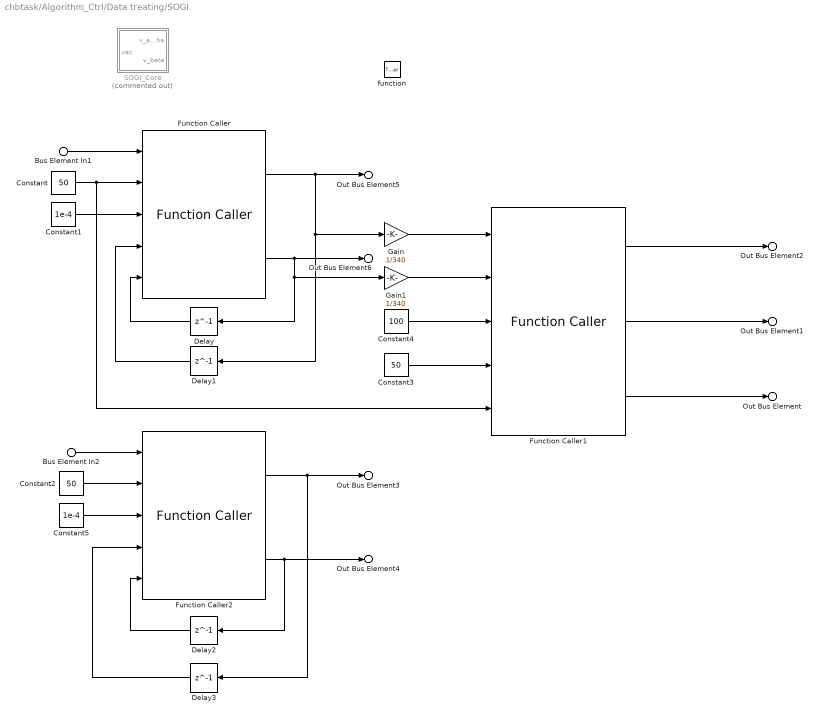
== system chbtask/Algorithm_Ctrl/Data treating/SOGI ==
  Bus Element In1 : Inport  PortName=Sampling  Element=AC_in.Vgrid
  Bus Element In2 : Inport  PortName=Sampling  Element=AC_in.Igrid
  function : TriggerPort  TriggerType=function-call  VariantControl=(inherit)
  Constant : Constant  Value=50  OutDataTypeStr=single
  Constant1 : Constant  Value=1e-4  OutDataTypeStr=single
  Constant2 : Constant  Value=50  OutDataTypeStr=single
  Constant3 : Constant  Value=50  OutDataTypeStr=single
  Constant4 : Constant  Value=100  OutDataTypeStr=single
  Constant5 : Constant  Value=1e-4  OutDataTypeStr=single
  Delay{,1..3} (4 alike) : Delay  DelayLength=1  InputProcessing=Columns as channels (frame based)
  Function Caller : FunctionCaller  FunctionPrototype=[alpha,beta] = Func.Sogi_ZOH(uk,freq,T,alpha1,beta1)  InputArgumentSpecifications=<Enter example>  OutputArgumentSpecifications=<Enter example>
  Function Caller1 : FunctionCaller  FunctionPrototype=[theta,cosine,sine] = Func.PLL(alpha,beta,Kp,Ki,freq)  InputArgumentSpecifications=<Enter example>  OutputArgumentSpecifications=<Enter example>
  Function Caller2 : FunctionCaller  FunctionPrototype=[alpha,beta] = Func.Sogi_ZOH(uk,freq,T,alpha1,beta1)  InputArgumentSpecifications=<Enter example>  OutputArgumentSpecifications=<Enter example>
  Gain : Gain  Gain=1/340
  Gain1 : Gain  Gain=1/340
  SOGI_Core : Stateflow chart  Commented=on  TreatAsAtomicUnit=on
  Out Bus Element1 : Outport  PortName=PLL  Element=cosin
  Out Bus Element : Outport  PortName=PLL  Element=sine
  Out Bus Element2 : Outport  PortName=PLL  Element=theta
  Out Bus Element3 : Outport  Port=2  PortName=Sogi_i  Element=alpha
  Out Bus Element4 : Outport  Port=2  PortName=Sogi_i  Element=beta
  Out Bus Element5 : Outport  Port=3  PortName=Sogi_v  Element=alpha
  Out Bus Element6 : Outport  Port=3  PortName=Sogi_v  Element=beta
  wires:
  Constant1/1 -> Function Caller/3
  Function Caller/2 -> Out Bus Element6/1, Delay/1, Gain1/1
  Delay/1 -> Function Caller/5
  Function Caller/1 -> Out Bus Element5/1, Delay1/1, Gain/1
  Delay1/1 -> Function Caller/4
  Constant4/1 -> Function Caller1/3
  Constant3/1 -> Function Caller1/4
  Constant/1 -> Function Caller/2, Function Caller1/5
  Gain/1 -> Function Caller1/1
  Gain1/1 -> Function Caller1/2
  Function Caller1/2 -> Out Bus Element1/1
  Function Caller1/3 -> Out Bus Element/1
  Function Caller1/1 -> Out Bus Element2/1
  Bus Element In1/1 -> Function Caller/1
  Bus Element In2/1 -> Function Caller2/1
  Constant5/1 -> Function Caller2/3
  Constant2/1 -> Function Caller2/2
  Delay2/1 -> Function Caller2/5
  Delay3/1 -> Function Caller2/4
  Function Caller2/2 -> Out Bus Element4/1, Delay2/1
  Function Caller2/1 -> Out Bus Element3/1, Delay3/1

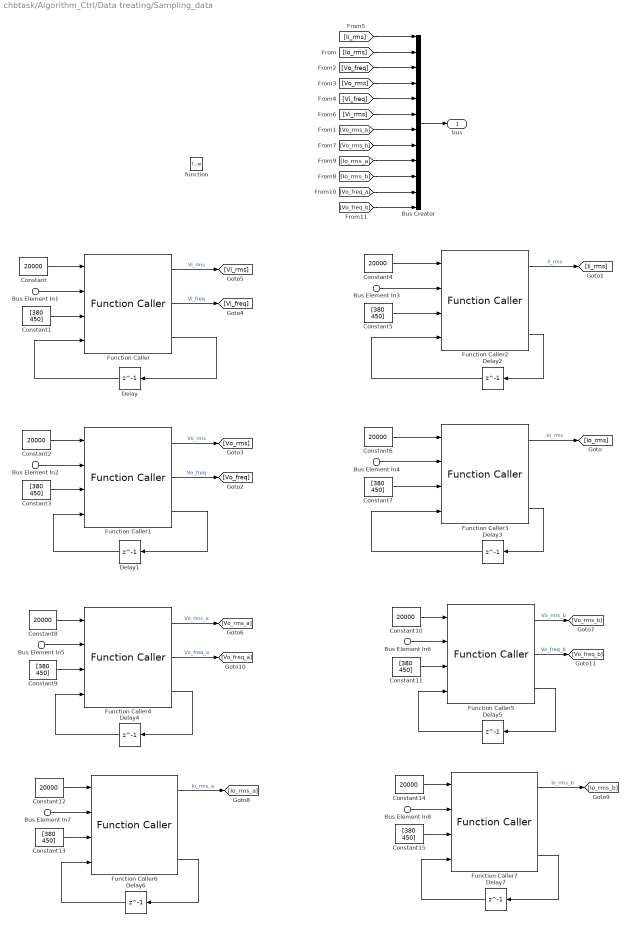
== system chbtask/Algorithm_Ctrl/Data treating/Sampling_data ==
  Bus Element In1 : Inport  PortName=Sampling  Element=AC_in.Vgrid
  Bus Element In3 : Inport  PortName=Sampling  Element=AC_in.Igrid
  Bus Element In2 : Inport  PortName=Sampling  Element=AC_out.Vgrid
  Bus Element In4 : Inport  PortName=Sampling  Element=AC_out.Igrid
  Bus Element In5 : Inport  PortName=Sampling  Element=AC_out_A.Vgrid
  Bus Element In7 : Inport  PortName=Sampling  Element=AC_out_A.Igrid
  Bus Element In6 : Inport  PortName=Sampling  Element=AC_out_B.Vgrid
  Bus Element In8 : Inport  PortName=Sampling  Element=AC_out_B.Igrid
  function : TriggerPort  TriggerType=function-call  VariantControl=(inherit)
  Bus Creator : BusCreator  Inputs=Ii_rms,Io_rms,Vo_freq,Vo_rms,Vi_freq,Vi_rms,Vo_rms_a,Vo_rms_b,Io_rms_a,Io_rms_b,Vo_freq_a,Vo_freq_b
  Constant{,2,4,6,8,10,12,14} (8 alike) : Constant  Value=20000  OutDataTypeStr=single
  Constant{1,3,5,7,9,11,13,15} (8 alike) : Constant  Value=[380 450]  OutDataTypeStr=single
  Delay{,1..7} (8 alike) : Delay  DelayLength=1  InitialCondition=[0 0 0 0 0]  InputProcessing=Columns as channels (frame based)
  Function Caller{,1..7} (8 alike) : FunctionCaller  FunctionPrototype=[X_rms,X_freq,out_data] = Func.Rms(Fs,X_data,limit_cnt,pre_data)  InputArgumentSpecifications=single(20000), single(0), single([380 450]), single([0 0 0 0 0])  OutputArgumentSpecifications=single(0), single(0), single([0 0 0 0 0])
  bus : Outport
  wires:
  Constant/1 -> Function Caller/1
  Function Caller/2 -> [Vi_freq]  "Vi_freq"
  Function Caller/1 -> [Vi_rms]  "Vi_rms"
  Constant1/1 -> Function Caller/3
  Delay/1 -> Function Caller/4
  Function Caller/3 -> Delay/1
  Constant2/1 -> Function Caller1/1
  Constant3/1 -> Function Caller1/3
  Function Caller1/3 -> Delay1/1
  Delay1/1 -> Function Caller1/4
  Function Caller1/2 -> [Vo_freq]  "Vo_freq"
  Function Caller1/1 -> [Vo_rms]  "Vo_rms"
  Bus Element In2/1 -> Function Caller1/2
  Bus Element In1/1 -> Function Caller/2
  Constant4/1 -> Function Caller2/1
  Constant5/1 -> Function Caller2/3
  Function Caller2/3 -> Delay2/1
  Delay2/1 -> Function Caller2/4
  Bus Element In3/1 -> Function Caller2/2
  Function Caller2/1 -> [Ii_rms]  "Ii_rms"
  Function Caller3/1 -> [Io_rms]  "Io_rms"
  Bus Element In4/1 -> Function Caller3/2
  Delay3/1 -> Function Caller3/4
  Function Caller3/3 -> Delay3/1
  Constant7/1 -> Function Caller3/3
  Constant6/1 -> Function Caller3/1
  [Ii_rms] -> Bus Creator/1
  [Io_rms] -> Bus Creator/2
  [Vo_freq] -> Bus Creator/3
  [Vo_rms] -> Bus Creator/4
  [Vi_freq] -> Bus Creator/5
  [Vi_rms] -> Bus Creator/6
  Bus Creator/1 -> bus/1
  Constant8/1 -> Function Caller4/1
  Constant9/1 -> Function Caller4/3
  Function Caller4/3 -> Delay4/1
  Delay4/1 -> Function Caller4/4
  Delay5/1 -> Function Caller5/4
  Function Caller5/3 -> Delay5/1
  Constant11/1 -> Function Caller5/3
  Constant10/1 -> Function Caller5/1
  Bus Element In6/1 -> Function Caller5/2
  Bus Element In5/1 -> Function Caller4/2
  Function Caller4/1 -> [Vo_rms_a]  "Vo_rms_a"
  Function Caller5/1 -> [Vo_rms_b]  "Vo_rms_b"
  [Vo_rms_a] -> Bus Creator/7
  [Vo_rms_b] -> Bus Creator/8
  Function Caller6/1 -> [Io_rms_a]  "Io_rms_a"
  Bus Element In7/1 -> Function Caller6/2
  Delay6/1 -> Function Caller6/4
  Function Caller6/3 -> Delay6/1
  Constant13/1 -> Function Caller6/3
  Constant12/1 -> Function Caller6/1
  Constant14/1 -> Function Caller7/1
  Constant15/1 -> Function Caller7/3
  Function Caller7/3 -> Delay7/1
  Delay7/1 -> Function Caller7/4
  Bus Element In8/1 -> Function Caller7/2
  Function Caller7/1 -> [Io_rms_b]  "Io_rms_b"
  [Io_rms_a] -> Bus Creator/9
  [Io_rms_b] -> Bus Creator/10
  Function Caller4/2 -> [Vo_freq_a]  "Vo_freq_a"
  Function Caller5/2 -> [Vo_freq_b]  "Vo_freq_b"
  [Vo_freq_a] -> Bus Creator/11
  [Vo_freq_b] -> Bus Creator/12

== system chbtask/Algorithm_Ctrl/MainCtrl/Subsystem ==
  stabflg : Inport  OutDataTypeStr=boolean
  CMD_Model : Inport  Port=2
  Chart : Stateflow chart  TreatAsAtomicUnit=on
  Out Bus Element : Outport  PortName=Relay
  wires:
  Chart/1(Relay) -> Out Bus Element/1
  CMD_Model/1 -> Chart/2(CMD_Model)
  stabflg/1 -> Chart/1(stabflg)

== system chbtask/Algorithm_Ctrl/MainCtrl/inv120_func ==
  En_INV120 : Inport
  Bus Element In2 : Inport  Port=2  PortName=Algorithm
  Bus Element In3 : Inport  Port=3  PortName=Sampling
  function : TriggerPort  TriggerType=function-call  VariantControl=(inherit)
  inv120_en : Subsystem
  duty : Outport  PortDimensions=[1 2]  VectorParamsAs1DForOutWhenUnconnected=off
  stabflg : Outport  Port=2  OutDataTypeStr=boolean
  wires:
  En_INV120/1 -> stabflg/1, inv120_en/Enable
  inv120_en/1(duty) -> duty/1
  Bus Element In2/1 -> inv120_en/1(Algorithm)
  Bus Element In3/1 -> inv120_en/2(Sampling)

== system chbtask/Algorithm_Ctrl/MainCtrl/inv240_func ==
  En_INV240 : Inport
  Bus Element In2 : Inport  Port=2  PortName=Algorithm
  function : TriggerPort  TriggerType=function-call  VariantControl=(inherit)
  inv240_en : Subsystem
  duty : Outport  PortDimensions=[1 2]
  stabflg : Outport  Port=2  OutDataTypeStr=boolean
  wires:
  inv240_en/1(duty) -> duty/1
  En_INV240/1 -> stabflg/1, inv240_en/Enable
  Bus Element In2/1 -> inv240_en/1(Algorithm)

== system chbtask/Algorithm_Ctrl/MainCtrl/pfc120_func ==
  EN_PCF120 : Inport
  Bus Element In2 : Inport  Port=2  PortName=PLL
  Bus Element In3 : Inport  Port=3  PortName=Sampling
  Bus Element In4 : Inport  Port=4  PortName=Algorithm
  function : TriggerPort  TriggerType=function-call  VariantControl=(inherit)
  Chart : Stateflow chart  TreatAsAtomicUnit=on
  pfc120_en : Subsystem
  duty : Outport  PortDimensions=[1 2]  VectorParamsAs1DForOutWhenUnconnected=off
  stabflg : Outport  Port=2  OutDataTypeStr=boolean
  wires:
  pfc120_en/1(duty) -> duty/1
  EN_PCF120/1 -> Chart/1(En_PFC120)
  Chart/1(run_en) -> pfc120_en/Enable, stabflg/1
  Bus Element In2/1 -> pfc120_en/1(PLL)
  Bus Element In3/1 -> pfc120_en/2(Sampling)
  Bus Element In4/1 -> pfc120_en/3(Algorithm)

== system chbtask/Algorithm_Ctrl/MainCtrl/pfc240_func ==
  En_PFC240 : Inport
  In Bus Element : Inport  Port=2  PortName=PLL
  Bus Element In3 : Inport  Port=3  PortName=Sampling
  Bus Element In4 : Inport  Port=4  PortName=Algorithm
  function : TriggerPort  TriggerType=function-call  VariantControl=(inherit)
  Chart : Stateflow chart  TreatAsAtomicUnit=on
  pfc240_en : Subsystem
  duty : Outport  PortDimensions=[1 2]
  stabflg : Outport  Port=2  OutDataTypeStr=boolean
  wires:
  pfc240_en/1(duty) -> duty/1
  In Bus Element/1 -> pfc240_en/1(PLL)
  En_PFC240/1 -> Chart/1(En_PFC240)
  Chart/1(run_en) -> stabflg/1, pfc240_en/Enable
  Bus Element In3/1 -> pfc240_en/2(Sampling)
  Bus Element In4/1 -> pfc240_en/3(Algorithm)

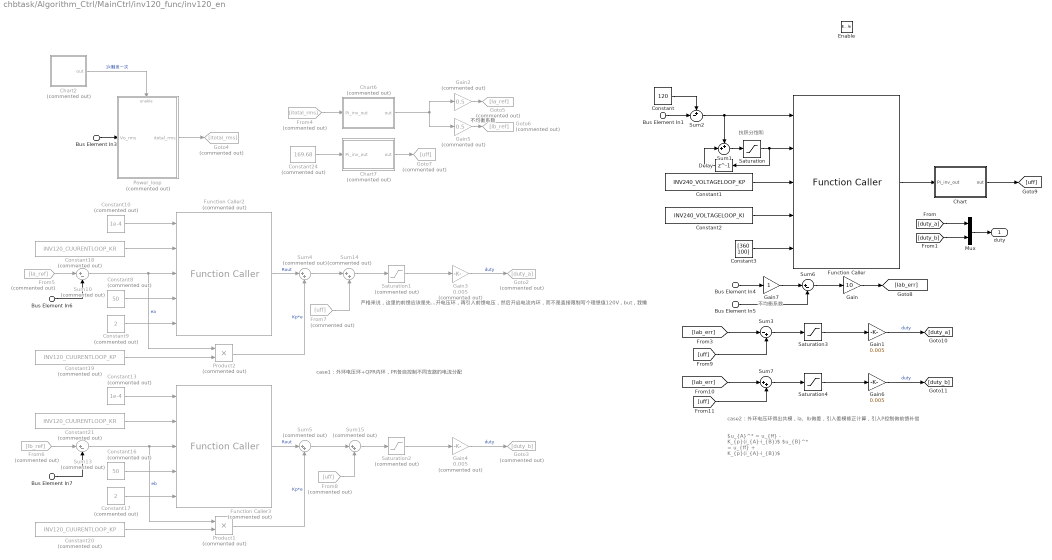
== system chbtask/Algorithm_Ctrl/MainCtrl/inv120_func/inv120_en ==
  note: 不均衡系数
  note: $u_{A}^* = u_{ff} - K_{p}(i_{A}-i_{B})$
      | $u_{B}^* = u_{ff} + K_{p}(i_{A}-i_{B})$
  note: case2：外环电压环得出共模，Ia、Ib做差，引入差模修正计算，引入P控制做前馈补偿
  note: case1：外环电压环+QPR内环，PR各自控制不同支路的电流分配
  note: 严格来说，这里的前馈应该是先开电压环，再引入前馈电压，然后开启电流内环，而不是直接限制写个理想值120V，but，我懒
  note: 不均衡系数
  note: 抗积分饱和
  Bus Element In3 : Inport  PortName=Algorithm  Element=B.Vo_rms
  Bus Element In1 : Inport  PortName=Algorithm  Element=A.Vo_rms
  Bus Element In6 : Inport  Port=2  PortName=Sampling  Element=AC_out_A.Igrid
  Bus Element In4 : Inport  Port=2  PortName=Sampling  Element=AC_out_A.Igrid
  Bus Element In7 : Inport  Port=2  PortName=Sampling  Element=AC_out_B.Igrid
  Bus Element In5 : Inport  Port=2  PortName=Sampling  Element=AC_out_B.Igrid
  Enable : EnablePort
  Chart : Stateflow chart  TreatAsAtomicUnit=on
  Chart2 : Stateflow chart  Commented=on  TreatAsAtomicUnit=on
  Chart6 : Stateflow chart  Commented=on  TreatAsAtomicUnit=on
  Chart7 : Stateflow chart  Commented=on  TreatAsAtomicUnit=on
  Constant : Constant  Value=120  OutDataTypeStr=single
  Constant1 : Constant  Value=INV240_VOLTAGELOOP_KP  OutDataTypeStr=single
  Constant10 : Constant  Commented=on  Value=1e-4  OutDataTypeStr=single
  Constant13 : Constant  Commented=on  Value=1e-4  OutDataTypeStr=single
  Constant16 : Constant  Commented=on  Value=50  OutDataTypeStr=single
  Constant17 : Constant  Commented=on  Value=2  OutDataTypeStr=single
  Constant18 : Constant  Commented=on  Value=INV120_CUURENTLOOP_KR  OutDataTypeStr=single
  Constant19 : Constant  Commented=on  Value=INV120_CUURENTLOOP_KP  OutDataTypeStr=single
  Constant2 : Constant  Value=INV240_VOLTAGELOOP_KI  OutDataTypeStr=single
  Constant20 : Constant  Commented=on  Value=INV120_CUURENTLOOP_KP  OutDataTypeStr=single
  Constant21 : Constant  Commented=on  Value=INV120_CUURENTLOOP_KR  OutDataTypeStr=single
  Constant24 : Constant  Commented=on  Value=169.68  OutDataTypeStr=single
  Constant3 : Constant  Value=[360 100]  OutDataTypeStr=single
  Constant8 : Constant  Commented=on  Value=50  OutDataTypeStr=single
  Constant9 : Constant  Commented=on  Value=2  OutDataTypeStr=single
  Delay : Delay  DelayLength=1  InputProcessing=Columns as channels (frame based)
  From4 : From  Commented=on  GotoTag=itotal_rms
  From5 : From  Commented=on  GotoTag=Ia_ref
  From6 : From  Commented=on  GotoTag=Ib_ref
  From7 : From  Commented=on  GotoTag=uff
  From8 : From  Commented=on  GotoTag=uff
  Function Caller : FunctionCaller  FunctionPrototype=PI_out = Func.PI_Ctrl(error,err_sum,Kp,Ki,out_limit)  InputArgumentSpecifications=<Enter example>  OutputArgumentSpecifications=<Enter example>
  Function Caller2 : FunctionCaller  Commented=on  FunctionPrototype=R_out = Func.R_Ctrl(Ts,Kr,uk,freq0,freqc)  InputArgumentSpecifications=<Enter example>  OutputArgumentSpecifications=<Enter example>
  Function Caller3 : FunctionCaller  Commented=on  FunctionPrototype=R_out = Func.R_Ctrl(Ts,Kr,uk,freq0,freqc)  InputArgumentSpecifications=<Enter example>  OutputArgumentSpecifications=<Enter example>
  Gain : Gain  Gain=10
  Gain1 : Gain  Gain=0.005  OutDataTypeStr=single
  Gain2 : Gain  Commented=on  Gain=0.5  OutDataTypeStr=single
  Gain3 : Gain  Commented=on  Gain=0.005  OutDataTypeStr=single
  Gain4 : Gain  Commented=on  Gain=0.005  OutDataTypeStr=single
  Gain5 : Gain  Commented=on  Gain=0.5  OutDataTypeStr=single
  Gain6 : Gain  Gain=0.005  OutDataTypeStr=single
  Gain7 : Gain
  Goto2 : Goto  Commented=on  GotoTag=duty_a
  Goto3 : Goto  Commented=on  GotoTag=duty_b
  Goto4 : Goto  Commented=on  GotoTag=itotal_rms
  Goto5 : Goto  Commented=on  GotoTag=Ia_ref
  Goto6 : Goto  Commented=on  GotoTag=Ib_ref
  Goto7 : Goto  Commented=on  GotoTag=uff
  Mux : Mux  Inputs=2
  Power_loop : Subsystem  Commented=on
  Product1 : Product  Commented=on
  Product2 : Product  Commented=on
  Saturation : Saturate  UpperLimit=190/INV240_VOLTAGELOOP_KI  LowerLimit=70/INV240_VOLTAGELOOP_KI
  Saturation1 : Saturate  Commented=on  UpperLimit=200  LowerLimit=-200  OutDataTypeStr=single
  Saturation2 : Saturate  Commented=on  UpperLimit=200  LowerLimit=-200  OutDataTypeStr=single
  Saturation3 : Saturate  UpperLimit=200  LowerLimit=-200  OutDataTypeStr=single
  Saturation4 : Saturate  UpperLimit=200  LowerLimit=-200  OutDataTypeStr=single
  Sum1 : Sum  Inputs=++|
  Sum10 : Sum  Commented=on  Inputs=|+-  OutDataTypeStr=single  AccumDataTypeStr=single
  Sum13 : Sum  Commented=on  Inputs=|+-
  Sum{4..5,14..15} (4 alike) : Sum  Commented=on  Inputs=|++  OutDataTypeStr=single  AccumDataTypeStr=single
  Sum2 : Sum  Inputs=+-|
  Sum3 : Sum  Inputs=|-+  OutDataTypeStr=single  AccumDataTypeStr=single
  Sum6 : Sum  Inputs=|+-
  Sum7 : Sum  Inputs=|++  OutDataTypeStr=single  AccumDataTypeStr=single
  duty : Outport  OutDataTypeStr=single  PortDimensions=[1 2]
  wires:
  [duty_b] -> Mux/2
  [duty_a] -> Mux/1
  Mux/1 -> duty/1
  Constant8/1 -> Function Caller2/4
  Constant9/1 -> Function Caller2/5
  Constant10/1 -> Function Caller2/1
  Chart2/1(out) -> Power_loop/Enable  "1k触发一次"
  Bus Element In3/1 -> Power_loop/1(Vo_rms)
  Constant13/1 -> Function Caller3/1
  Constant17/1 -> Function Caller3/5
  Constant16/1 -> Function Caller3/4
  Power_loop/1(itotal_rms) -> Goto4/1
  From4/1 -> Chart6/1(Pi_inv_out)
  Chart6/1(out) -> Gain5/1, Gain2/1
  Sum10/1 -> Product2/1, Function Caller2/3  "ea"
  From5/1 -> Sum10/1
  Bus Element In6/1 -> Sum10/2
  From6/1 -> Sum13/1
  Bus Element In7/1 -> Sum13/2
  Sum13/1 -> Product1/1, Function Caller3/3  "eb"
  Saturation1/1 -> Gain3/1
  Saturation2/1 -> Gain4/1
  Gain4/1 -> Goto3/1  "duty"
  Gain3/1 -> Goto2/1  "duty"
  Constant24/1 -> Chart7/1(Pi_inv_out)
  Chart7/1(out) -> Goto7/1
  Sum15/1 -> Saturation2/1
  Sum14/1 -> Saturation1/1
  From7/1 -> Sum14/2
  From8/1 -> Sum15/2
  Gain2/1 -> Goto5/1
  Gain5/1 -> Goto6/1
  Constant19/1 -> Product2/2
  Constant18/1 -> Function Caller2/2
  Constant20/1 -> Product1/2
  Constant21/1 -> Function Caller3/2
  Bus Element In5/1 -> Sum6/2
  Sum6/1 -> Gain/1
  Gain/1 -> [Iab_err]
  Sum4/1 -> Sum14/1
  Sum5/1 -> Sum15/1
  Function Caller2/1 -> Sum4/1  "Rout"
  Product2/1 -> Sum4/2  "Kp*e"
  Function Caller3/1 -> Sum5/1  "Rout"
  Product1/1 -> Sum5/2  "Kp*e"
  Saturation/1 -> Delay/1, Function Caller/2
  Sum2/1 -> Sum1/1, Function Caller/1
  Constant1/1 -> Function Caller/3
  Constant2/1 -> Function Caller/4
  Sum1/1 -> Saturation/1
  Delay/1 -> Sum1/2
  Function Caller/1 -> Chart/1(Pi_inv_out)
  Constant3/1 -> Function Caller/5
  Bus Element In1/1 -> Sum2/2
  Constant/1 -> Sum2/1
  Chart/1(out) -> [uff]
  [Iab_err] -> Sum3/1
  Gain1/1 -> [duty_a]  "duty"
  [uff] -> Sum3/2
  Sum3/1 -> Saturation3/1
  Saturation3/1 -> Gain1/1
  Saturation4/1 -> Gain6/1
  Sum7/1 -> Saturation4/1
  [uff] -> Sum7/2
  Gain6/1 -> [duty_b]  "duty"
  [Iab_err] -> Sum7/1
  Bus Element In4/1 -> Gain7/1
  Gain7/1 -> Sum6/1
